simulink model "sm_car"  (R2025a)
settings: Solver=ode23t  StartTime=0.0  StopTime=400  MaxStep=0.4  RelTol=1e-3  AbsTol=1e-3  EnableMultiTasking=on
PreLoadFcn:
  | % Due to usability issue in Repeating Sequence block
  | warning('off','Simulink:Masking:Invalid');
  | 
  | % Eliminate unnecessary warnings in inactive variants
  | % Warnings generated only if you click through inactive variant
  | warning('off','MATLAB:nonExistentField');
  | warning('off','Simulink:Parameters:BlkParamUndefined');
PostLoadFcn:
  | set_param([bdroot '/Vehicle'],'popup_trailer','Off')
  | warning('off','sm:sli:setup:compile:LocalSolverNotSupported')
  | %sm_car_config_maneuver(bdroot,'WOT Braking');
  | sm_car_config_vehicle(bdroot,'false');
  | sm_car_config_logging(bdroot);
InitFcn:
  | sm_car_config_camera;
  | Vehicle = sm_car_vehcfg_checkConfig(Vehicle);
  | sm_car_check_tire_model(bdroot);
StartFcn:
  | tic;
StopFcn:
  | Elapsed_Sim_Time = toc;
  | % disp(['Elapsed Sim Time = ' num2str(Elapsed_Sim_Time)]);
undefined symbols (not defined in the file): Axle1D, AxleIn, Camera, Control, Driver, Free, Init, Maneuver, Pedal, RaceFix, RaceSpin, Scene, ShaftL1, ShaftL2, ShaftR1, ShaftR2, Soft, Stiff, Visual, X, xy_data_car_side, Y, Z
libraries: sm_lib x1546, nesl_utility x528, fl_lib x480, SimscapeFluids_lib x61, sdl_lib x49, simulink x29, ee_lib x7, simulink_extras x6, Linkage_Systems x4, Tire_1x2x x4, AntiRollBar_Systems x2, Linkage_Decoupled x2
(part 5 of 79)

== system sm_car/Controller/TrqVec 4Motor/Power_TqVec ==
  In Bus Element6 : Inport  PortName=DrvBus  Element=rAccelPedal
  In Bus Element2 : Inport  PortName=DrvBus  Element=aSteerWheel
  In Bus Element3 : Inport  PortName=DrvBus  Element=rBrakePedal
  In Bus Element : Inport  Port=2  PortName=VehBus  Element=Chassis.Body.CG.vx
  In Bus Element1 : Inport  Port=2  PortName=VehBus  Element=Power.MotorL2.w
  In Bus Element8 : Inport  Port=2  PortName=VehBus  Element=Power.MotorR2.w
  In Bus Element5 : Inport  Port=2  PortName=VehBus  Element=World.nYaw
  Bus Creator : BusCreator  Inputs=5
  Constant : Constant  Value=Control.trq_ratio_front
  Constant2 : Constant  Value=1-Control.trq_ratio_front
  Gain1 : Gain  Gain=1600
  Gain3 : Gain  Gain=0.5
  Gain4 : Gain  Gain=0.5
  Product : Product
  Product1 : Product
  Rate Limiter : RateLimiter  RisingSlewLimit=300  FallingSlewLimit=-5000  SampleTimeMode=inherited
  Torque Vectoring : Subsystem  mask(Torque Vectoring, Rear Wheels){vx_enable=Control.vx_enable, aSteerWheel_enable=Control.aSteerWheel_enable, aStr_to_aWhl=Control.aStr_to_aWhl, max_torque_delta=Control.max_torque_delta, P=Control.pGain, I=Control.iGain}
      mask prompts: vx_enable "Speed to enable (m/s)"; aSteerWheel_enable "Steering wheel angle to enable (rad)"; aStr_to_aWhl "Steering Ratio (Wheel/Steering Wheel)"; max_torque_delta "Max Torque Split (N*m)"; P "Simulink:masks:ProportionalP_MP"; I "Simulink:masks:IntegralI_MP"
      mask help: Basic torque vectoring algorithm which applies opposing offsets to the commanded torque of the rear wheels based on the error between the vehicle slip angle and the angle of the steered wheels.
      mask TypeOptions vx_enable: Enable/Enable vx/const
      mask TypeOptions aSteerWheel_enable: Enable/const/Value
      mask TypeOptions aStr_to_aWhl:
      | Vehicle Slip Angle Error/Steering Wheel
      | to Driving Wheel/Gain
      mask TypeOptions max_torque_delta: Max Delta Torque/Value
      mask TypeOptions P: PID Controller/P
      mask TypeOptions I: PID Controller/I
      mask DialogControl P Prompt: Proportional (P):
      mask DialogControl I Prompt: Integral (I):
  Power : Outport  VectorParamsAs1DForOutWhenUnconnected=off
  wires:
  Torque Vectoring/2(trqR2) -> Bus Creator/5  "MMotorR2Demand"
  Torque Vectoring/1(trqL2) -> Bus Creator/4  "MMotorL2Demand"
  In Bus Element3/1 -> Torque Vectoring/7(rBrake)
  In Bus Element5/1 -> Torque Vectoring/6(nYaw)
  In Bus Element8/1 -> Torque Vectoring/5(wR2)
  In Bus Element1/1 -> Torque Vectoring/4(wL2)
  In Bus Element2/1 -> Torque Vectoring/3(aSteerWheel)
  In Bus Element/1 -> Torque Vectoring/2(vx)
  Product1/1 -> Torque Vectoring/1(trqA2)
  Bus Creator/1 -> Power/1  "Power"
  Gain4/1 -> Bus Creator/3  "MMotorR1Demand"
  Gain3/1 -> Bus Creator/2  "MMotorL1Demand"
  Product/1 -> Gain4/1, Gain3/1, Bus Creator/1  "MMotorA1Demand"
  Constant2/1 -> Product1/2
  Constant/1 -> Product/1
  Rate Limiter/1 -> Product/2, Product1/1
  In Bus Element6/1 -> Gain1/1
  Gain1/1 -> Rate Limiter/1

== system sm_car/Controller/TrqVec 4Motor/Spring Control ==
  VehBus : Inport
  In Bus Element : Inport  Port=2  PortName=Ctrl  Element=Axle1
  In Bus Element1 : Inport  Port=2  PortName=Ctrl  Element=Axle2
  Bus Creator : BusCreator  Inputs=4
  Bus Selector : BusSelector  OutputSignals=Chassis.Damper.L1,Chassis.Damper.R1,Chassis.Damper.L2,Chassis.Damper.R2
  Spring Control A1 : Subsystem  Variant=on  VariantControlMode=label  VariantControl=Choice  LabelModeActiveChoice=None  mask(Spring Control, One Axle){popup_spring_control=None, popup_gas_spring=Stiff}
      mask prompts: popup_spring_control "Spring Control"; popup_gas_spring "Gas Spring"
      mask help: Configurable spring control for left and right sides.
      mask init:
      | bh = gcb;
      | set_param(bh,'LabelModeActiveChoice',get_param(bh,'popup_spring_control'));
      | set_param([bh '/Hydropneumatic'],'popup_gas_spring',get_param(bh,'popup_gas_spring'));
      mask TypeOptions popup_spring_control: None | Hydropneumatic
      mask Callback popup_spring_control:
      | bh = gcb;
      | maskObj = Simulink.Mask.get(bh); % Get the mask object of the current block
      | psg_h   = maskObj.getParameter('popup_gas_spring'); % Get the parameter to hide
      | 
      | % Check the value of ControlParam
      | controlParamValue = get_param(bh, 'popup_spring_control');
      | 
      | psg_h.Visible  = 'off';
      | 
      | if strcmp(controlParamValue, 'Hydropneumatic')
      |     psg_h.Visible  = 'on';
      | else
      |     psg_h.Visible  = 'off';
      | end
      mask TypeOptions popup_gas_spring: Stiff | Soft
      mask Display: disp(' ')
  Spring Control A2 : Subsystem  Variant=on  VariantControlMode=label  VariantControl=Choice  LabelModeActiveChoice=None  mask(Spring Control, One Axle){popup_spring_control=None, popup_gas_spring=Stiff}
      mask prompts: popup_spring_control "Spring Control"; popup_gas_spring "Gas Spring"
      mask help: Configurable spring control for left and right sides.
      mask init:
      | bh = gcb;
      | set_param(bh,'LabelModeActiveChoice',get_param(bh,'popup_spring_control'));
      | set_param([bh '/Hydropneumatic'],'popup_gas_spring',get_param(bh,'popup_gas_spring'));
      mask TypeOptions popup_spring_control: None | Hydropneumatic
      mask Callback popup_spring_control:
      | bh = gcb;
      | maskObj = Simulink.Mask.get(bh); % Get the mask object of the current block
      | psg_h   = maskObj.getParameter('popup_gas_spring'); % Get the parameter to hide
      | 
      | % Check the value of ControlParam
      | controlParamValue = get_param(bh, 'popup_spring_control');
      | 
      | psg_h.Visible  = 'off';
      | 
      | if strcmp(controlParamValue, 'Hydropneumatic')
      |     psg_h.Visible  = 'on';
      | else
      |     psg_h.Visible  = 'off';
      | end
      mask TypeOptions popup_gas_spring: Stiff | Soft
      mask Display: disp(' ')
  Spring : Outport
  wires:
  VehBus/1 -> Bus Selector/1
  Spring Control A1/1(L) -> Bus Creator/1  "L1"
  Bus Selector/1 -> Spring Control A1/1(mL)  "<L1>"
  Bus Selector/2 -> Spring Control A1/2(mR)  "<R1>"
  Bus Selector/3 -> Spring Control A2/1(mL)  "<L2>"
  Bus Selector/4 -> Spring Control A2/2(mR)  "<R2>"
  Bus Creator/1 -> Spring/1  "Spring"
  Spring Control A1/2(R) -> Bus Creator/2  "R1"
  Spring Control A2/1(L) -> Bus Creator/3  "L2"
  Spring Control A2/2(R) -> Bus Creator/4  "R2"
  In Bus Element/1 -> Spring Control A1/3(Inp)
  In Bus Element1/1 -> Spring Control A2/3(Inp)

== system sm_car/Controller/TrqVec 4Motor/Susp ==
  aSteerWheel : Inport
  vx : Inport  Port=2
  Bus Creator1 : BusCreator  Inputs=1
  Bus Creator3 : BusCreator  Inputs=1
  Steer Axle 1 : Subsystem
  Steer Axle 2 : Subsystem
  SuspA1 : Outport  VectorParamsAs1DForOutWhenUnconnected=off
  SuspA2 : Outport  Port=2  VectorParamsAs1DForOutWhenUnconnected=off
  wires:
  Steer Axle 2/1(Steer) -> Bus Creator3/1
  Bus Creator1/1 -> SuspA1/1  "SuspA1"
  Steer Axle 1/1(Steer) -> Bus Creator1/1
  aSteerWheel/1 -> Steer Axle 1/1(aSteerWheel), Steer Axle 2/1(aSteerWheel)  "aSteerWheel"
  Bus Creator3/1 -> SuspA2/1  "SuspA2"
  vx/1 -> Steer Axle 2/2(vx), Steer Axle 1/2(vx)

== system sm_car/Driver/Closed Loop/Driver ==
  vx : Inport
  Ref : Inport  Port=2
  CurPose : Inport  Port=3
  Preview : Inport  Port=4
  Bus Creator5 : BusCreator  Inputs=4
  Bus Selector1 : BusSelector  OutputSignals=vTarget
  Bus Selector2 : BusSelector  OutputSignals=dist
  Constant9 : Constant  Value=0
  Cur Pose : Subsystem
  Filter Steer Cmd : TransferFcn  Denominator=[1/Driver.Lateral.fSteerCutoff.Value 1]
  Fwd Rev : Subsystem
  Lateral Driver : Subsystem  Variant=on  VariantControlMode=label  VariantControl=Choice  LabelModeActiveChoice=Stanley  mask{Lateral=Driver.Lateral, VariantLabel=Driver.Lateral.class.Value}
      mask prompts: Lateral "Lateral Driver Parameters (structure)"; VariantLabel "Variant Label"
      mask init:
      | curblk = gcb;
      | 
      | % Set variant for this block 
      | set_param(curblk,'LabelModeActiveChoice',VariantLabel);
  Longitudinal Driver : Subsystem  mask(Longitudinal Driver (Velocity-tracking Controller)){SPEED_LOOKAHEAD_TIME=Driver.Long.FFLookahead.Value, C_ROLLING_RESISTANCE_COEFF=Driver.Long.NRollingResistance.Value, ROAD_FRICTION_COEFF=Driver.Long.NRoadFriction.Value, mVehicle=Driver.Long.mVehicle.Value, gGravity=Driver.Long.gGravity.Value, FTractive=Driver.Long.FTractive.Value, KP_SPEED=Driver.Long.Kp.Value, KI_SPEED=Driver.Long.Ki.Value, MAX_ACCEL_MPS2=Driver.Long.gMaxAccel.Value, MAX_DECEL_MPS2=Driver.Long.gMaxDecel.Value, Cdrag=Vehicle.Chassis.Aero.CD.Value, rho_air=Vehicle.Chassis.Aero.rho_air.Value, ARef=Vehicle.Chassis.Aero.ARef.Value}
      mask prompts: SPEED_LOOKAHEAD_TIME "Lookahead time (s)"; C_ROLLING_RESISTANCE_COEFF "Rolling resistance coefficient"; ROAD_FRICTION_COEFF "Road friction coefficient"; mVehicle "Total Vehicle mass (kg)"; gGravity "Gravity (m/s)"; FTractive "Tractive Force (N)"; KP_SPEED "Proportional gain, Kp"; KI_SPEED "Integral gain, Ki"; MAX_ACCEL_MPS2 "Max acceleration (m/s^2, positive number))"; MAX_DECEL_MPS2 "Max deceleration (m/s^2, must be negative)"; Cdrag "Drag coefficient"; rho_air "Density of air (kg/m^3)"; ARef "Frontal Area (m^2)"
      mask help: Implements a PI controller with feedforward for velocity tracking.
      mask DialogControl cont_feedforward Prompt: Feed-Forward Controller parameters
      mask DialogControl cont_feedback Prompt: Feedback Controller parameters
      mask DialogControl cont_drag Prompt: Drag
  Ref Pose and Distance : Subsystem
  Transfer Fcn : TransferFcn  Denominator=[1/(Driver.Long.fAccelCutoff.Value) 1]
  Transfer Fcn1 : TransferFcn  Denominator=[1/(Driver.Long.fBrakeCutoff.Value) 1]
  DrvBus : Outport  VectorParamsAs1DForOutWhenUnconnected=off
  wires:
  Bus Selector2/1 -> Longitudinal Driver/4(Distance)  "<dist>"
  Fwd Rev/2(vxFwRv) -> Longitudinal Driver/3(vx)
  Bus Selector1/1 -> Fwd Rev/2(vT)  "<vTarget>"
  Ref Pose and Distance/2(Dist) -> Lateral Driver/2(Distance)
  Preview/1 -> Longitudinal Driver/1(Preview), Lateral Driver/5(Preview)
  Lateral Driver/1(steeringAngle) -> Filter Steer Cmd/1
  Fwd Rev/1(dir) -> Longitudinal Driver/2(dir), Lateral Driver/6(Direction)
  vx/1 -> Fwd Rev/1(vx), Lateral Driver/4(v_x)
  Cur Pose/1(CurPose) -> Lateral Driver/3(currentPose)
  CurPose/1 -> Cur Pose/1(Cur)
  Constant9/1 -> Longitudinal Driver/5(current_slope_rad)
  Bus Creator5/1 -> DrvBus/1  "DrvBus"
  Longitudinal Driver/1(AccelCmd) -> Transfer Fcn/1
  Longitudinal Driver/2(DecelCmd) -> Transfer Fcn1/1
  Transfer Fcn1/1 -> Bus Creator5/4  "rBrakePedal"
  Transfer Fcn/1 -> Bus Creator5/3  "rAccelPedal"
  Ref/1 -> Bus Creator5/1, Bus Selector2/1, Bus Selector1/1, Ref Pose and Distance/1(Ref)
  Ref Pose and Distance/1(RefPose) -> Lateral Driver/1(referencePose)
  Filter Steer Cmd/1 -> Bus Creator5/2  "aSteerWheel"

== system sm_car/Driver/Closed Loop/Driver Override ==
  In : Inport
  None : Subsystem  VariantControl=None
  Override : Subsystem  VariantControl=Override
  DrvBus : Outport

== system sm_car/Driver/Closed Loop/Maneuver ==
  note: Fwd or
      | Rev
  VehBus : Inport
  Override : Inport  Port=2
  Abs : Abs  ZeroCross=off  SaturateOnIntegerOverflow=off
  Bus Creator : BusCreator  Inputs=7
  Bus Creator1 : BusCreator  Inputs=5
  Bus Selector : BusSelector  OutputSignals=World.x,World.y,World.z,World.aRoll,World.aPitch,World.aYaw,Chassis.Body.CG.vx
  Bus Selector1 : BusSelector  OutputSignals=x,y,z,vx
  Bus Selector2 : BusSelector  OutputSignals=Chassis.Body.CG.vx
  Bus Selector3 : BusSelector  OutputSignals=y,x,nLap,ayaw
  Constant : Constant  Value=-1
  Constant6 : Constant  Value=Maneuver.Trajectory.xTrajectory.Value
  Constant8 : Constant  Value=Maneuver.Trajectory.aYaw.Value
  Count Lap : Subsystem
  MATLAB Function : MATLAB Function  SystemSampleTime=0.1  mask{nPreviewPoints=Maneuver.nPreviewPoints.Value}
      mask prompts: nPreviewPoints "Number of Preview Points"
  Max Lateral Distance (m) : Constant  Value=Maneuver.xMaxLat.Value
  Memory : Memory  InitialCondition=-1
  Min Target Speed (m/s) : Constant  Value=Maneuver.vMinTarget.Value
  Mux : Mux  Inputs=3
  Mux1 : Mux  Inputs=3
  PoseTarget Visual : Subsystem
  Switch : Switch  Criteria=u2 > Threshold  SaturateOnIntegerOverflow=off  InputSameDT=off
  Target Speed Gain : Constant  Value=Maneuver.vGain.Value
  Window of Points to Check : Constant  Value=10
  preview distance : Lookup_n-D  NumberOfTableDimensions=1  BreakpointsForDimension1=Maneuver.xPreview.v.Value  Table=Maneuver.xPreview.x.Value  InternalRulePriority=Speed  RndMeth=Simplest
  vx override : Subsystem
  window only : Constant  Value=0
  x override : Subsystem
  y override : Subsystem
  z override : Subsystem
  vx : Outport  VectorParamsAs1DForOutWhenUnconnected=off
  Ref : Outport  Port=2  VectorParamsAs1DForOutWhenUnconnected=off
  CurPose : Outport  Port=3  VectorParamsAs1DForOutWhenUnconnected=off
  Preview : Outport  Port=4  VectorParamsAs1DForOutWhenUnconnected=off
  simres : Outport  Port=5  VectorParamsAs1DForOutWhenUnconnected=off
  wires:
  MATLAB Function/14(pp_preview_speed_pts) -> Bus Creator1/5  "pp_preview_speed_pts"
  MATLAB Function/1(ref_z) -> PoseTarget Visual/1(ref_z)
  Bus Selector3/4 -> PoseTarget Visual/5(ref_ayaw)  "<ayaw>"
  Bus Selector3/3 -> PoseTarget Visual/4(Lap Count)  "<nLap>"
  Bus Selector3/2 -> PoseTarget Visual/3(ref_x)  "<x>"
  Bus Selector3/1 -> PoseTarget Visual/2(ref_y)  "<y>"
  Count Lap/1(lapC) -> Bus Creator/1  "nLap"
  Bus Selector2/1 -> vx/1  "<vx>"
  VehBus/1 -> Bus Selector/1, Bus Selector2/1
  Bus Creator1/1 -> Preview/1  "lookahead"
  MATLAB Function/13(pp_preview_dist_pts) -> Bus Creator1/4  "pp_preview_dist_pts"
  MATLAB Function/12(pp_preview_yaw_pts) -> Bus Creator1/3  "pp_preview_yaw_pts"
  MATLAB Function/11(pp_preview_y_pts) -> Bus Creator1/2  "pp_preview_y_pts"
  MATLAB Function/10(pp_preview_x_pts) -> Bus Creator1/1  "pp_preview_x_pts"
  MATLAB Function/7(ld) -> Bus Creator/7  "latdev"
  Min Target Speed (m/s)/1 -> MATLAB Function/12(minSpd)
  Target Speed Gain/1 -> MATLAB Function/13(speedGain)
  Max Lateral Distance (m)/1 -> MATLAB Function/11(maxld)
  Bus Selector/1 -> Mux/1  "<x>"
  Bus Selector/6 -> Mux1/3  "<aYaw>"
  Bus Selector/4 -> Mux1/1  "<aRoll>"
  Constant8/1 -> MATLAB Function/8(yaw)
  Bus Selector/7 -> Abs/1  "<vx>"
  Mux1/1 -> MATLAB Function/2(q)
  Bus Selector/5 -> Mux1/2  "<aPitch>"
  Constant6/1 -> MATLAB Function/9(dist)
  Mux/1 -> MATLAB Function/1(p)
  Bus Selector/3 -> Mux/3  "<z>"
  y override/1(y_ovr) -> MATLAB Function/4(posy)
  Bus Selector/2 -> Mux/2  "<y>"
  MATLAB Function/3(ref_x) -> Bus Creator/3  "x"
  x override/1(x_ovr) -> MATLAB Function/3(posx)
  MATLAB Function/8(cp) -> CurPose/1  "CurPose"
  preview distance/1 -> MATLAB Function/10(pd)
  MATLAB Function/4(ref_y) -> Bus Creator/4  "y"
  MATLAB Function/5(ref_ayaw) -> Bus Creator/5  "ayaw"
  MATLAB Function/2(ad) -> Count Lap/1(ad), Bus Creator/2  "dist"
  Bus Creator/1 -> Bus Selector3/1, Ref/1  "Reference"
  MATLAB Function/6(vTarget) -> Bus Creator/6  "vTarget"
  MATLAB Function/9(simres) -> simres/1
  Window of Points to Check/1 -> MATLAB Function/7(xywin)
  MATLAB Function/15(idx_ptMin) -> Memory/1
  Switch/1 -> MATLAB Function/14(idx_ptMin_prev)
  Constant/1 -> Switch/3
  window only/1 -> Switch/2
  Memory/1 -> Switch/1
  z override/1(z_ovr) -> MATLAB Function/5(posz)
  Override/1 -> Bus Selector1/1
  Bus Selector1/4 -> vx override/1(vx)  "<vx>"
  vx override/1(vx_ovr) -> MATLAB Function/6(speed)
  Bus Selector1/3 -> z override/1(z)  "<z>"
  Bus Selector1/2 -> y override/1(y)  "<y>"
  Bus Selector1/1 -> x override/1(x)  "<x>"
  Abs/1 -> preview distance/1

== system sm_car/Driver/Closed Loop/Override ==
  "dist " : Inport
  "Obs " : Inport  Port=2
  None : Subsystem  VariantControl=None  mask(No Driver Override){override=Scene.Mallory_Park_Obstacle.Override}
      mask prompts: override "Override parameters (structure)"
      mask help: Driver commands are not overridden, regardless of inputs to subsystem.
  " Ovr" : Outport  VectorParamsAs1DForOutWhenUnconnected=off

== system sm_car/Driver/Closed Loop/Scopes ==
  <vx> : Inport
  Ref : Inport  Port=2
  CurPose : Inport  Port=3
  DrvBus : Inport  Port=4
  Bus Selector : BusSelector  OutputSignals=vTarget
  Bus Selector1 : BusSelector  OutputSignals=aSteerWheel,rAccelPedal,rBrakePedal
  Compare vx to Target : Scope  NumInputPorts=2
      settings: ActiveDisplayYMinimum=-4.79181  ActiveDisplayYMaximum=0.54534
  RefPose : Scope
      settings: ActiveDisplayYMinimum=-598.75829  ActiveDisplayYMaximum=469.37365
  Scope1 : Scope  NumInputPorts=3
      settings: ActiveDisplayYMinimum=-1.19495  ActiveDisplayYMaximum=0.13277  DataLoggingVariableName=ScopeData2
  wires:
  DrvBus/1 -> Bus Selector1/1
  Bus Selector1/1 -> Scope1/1  "<aSteerWheel>"
  Bus Selector1/2 -> Scope1/2  "<rAccelPedal>"
  <vx>/1 -> Compare vx to Target/1
  Bus Selector1/3 -> Scope1/3  "<rBrakePedal>"
  CurPose/1 -> RefPose/1
  Bus Selector/1 -> Compare vx to Target/2  "<vTarget>"
  Ref/1 -> Bus Selector/1

== system sm_car/Driver/Open Loop/Open Loop ==
  Bus Creator : BusCreator  Inputs=7
  Bus Creator5 : BusCreator  Inputs=4
  Constant : Constant  Value=10000
  Constant{1..6} (6 alike) : Constant  Value=0
  Input Sequence Accel Pedal : simulink/Sources/Repeating Sequence  rep_seq_t=Maneuver.Accel.t.Value  rep_seq_y=Maneuver.Accel.rPedal.Value
  Input Sequence Brake Pedal : simulink/Sources/Repeating Sequence  rep_seq_t=Maneuver.Brake.t.Value  rep_seq_y=Maneuver.Brake.rPedal.Value
  "Input Sequence Steering Wheel " : simulink/Sources/Repeating Sequence  rep_seq_t=Maneuver.Steer.t.Value  rep_seq_y=Maneuver.Steer.aWheel.Value
  DrvBus : Outport  VectorParamsAs1DForOutWhenUnconnected=off
  wires:
  Constant6/1 -> Bus Creator/7  "nLap"
  Constant/1 -> Bus Creator/1  "dist"
  Bus Creator/1 -> Bus Creator5/1  "Reference"
  Constant4/1 -> Bus Creator/5  "vTarget"
  Constant3/1 -> Bus Creator/4  "ayaw"
  Constant2/1 -> Bus Creator/3  "y"
  Constant5/1 -> Bus Creator/6  "latdev"
  Constant1/1 -> Bus Creator/2  "x"
  Input Sequence Accel Pedal/1 -> Bus Creator5/3  "rAccelPedal"
  "Input Sequence Steering Wheel "/1 -> Bus Creator5/2  "aSteerWheel"
  Input Sequence Brake Pedal/1 -> Bus Creator5/4  "rBrakePedal"
  Bus Creator5/1 -> DrvBus/1  "DrvBus"

== system sm_car/Road/Mu Scaling by Position/Scaling factors FL ==
  muX : Inport
  muY : Inport  Port=2
  s_LKX : Constant  Value=LKX
  s_LKY : Constant  Value=LKY
  s_LKYC : Constant  Value=LKYC
  s_LKZC : Constant  Value=LKZC
  s_LTR : Constant  Value=LTR
  scaling_vector : Mux  Inputs=7
  scaling : Outport  VectorParamsAs1DForOutWhenUnconnected=off
  wires:
  muX/1 -> scaling_vector/1
  s_LKX/1 -> scaling_vector/2
  muY/1 -> scaling_vector/3
  s_LKY/1 -> scaling_vector/4
  s_LKYC/1 -> scaling_vector/5
  s_LTR/1 -> scaling_vector/6
  s_LKZC/1 -> scaling_vector/7
  scaling_vector/1 -> scaling/1

== system sm_car/Road/Mu Scaling by Position/Scaling factors FR ==
  muX : Inport
  muY : Inport  Port=2
  s_LKX : Constant  Value=LKX
  s_LKY : Constant  Value=LKY
  s_LKYC : Constant  Value=LKYC
  s_LKZC : Constant  Value=LKZC
  s_LTR : Constant  Value=LTR
  scaling_vector : Mux  Inputs=7
  scaling : Outport  VectorParamsAs1DForOutWhenUnconnected=off
  wires:
  muX/1 -> scaling_vector/1
  s_LKX/1 -> scaling_vector/2
  muY/1 -> scaling_vector/3
  s_LKY/1 -> scaling_vector/4
  s_LKYC/1 -> scaling_vector/5
  s_LTR/1 -> scaling_vector/6
  s_LKZC/1 -> scaling_vector/7
  scaling_vector/1 -> scaling/1

== system sm_car/Road/Mu Scaling by Position/Scaling factors RL ==
  muX : Inport
  muY : Inport  Port=2
  s_LKX : Constant  Value=LKX
  s_LKY : Constant  Value=LKY
  s_LKYC : Constant  Value=LKYC
  s_LKZC : Constant  Value=LKZC
  s_LTR : Constant  Value=LTR
  scaling_vector : Mux  Inputs=7
  scaling : Outport  VectorParamsAs1DForOutWhenUnconnected=off
  wires:
  muX/1 -> scaling_vector/1
  s_LKX/1 -> scaling_vector/2
  muY/1 -> scaling_vector/3
  s_LKY/1 -> scaling_vector/4
  s_LKYC/1 -> scaling_vector/5
  s_LTR/1 -> scaling_vector/6
  s_LKZC/1 -> scaling_vector/7
  scaling_vector/1 -> scaling/1

== system sm_car/Road/Mu Scaling by Position/Scaling factors RR ==
  muX : Inport
  muY : Inport  Port=2
  s_LKX : Constant  Value=LKX
  s_LKY : Constant  Value=LKY
  s_LKYC : Constant  Value=LKYC
  s_LKZC : Constant  Value=LKZC
  s_LTR : Constant  Value=LTR
  scaling_vector : Mux  Inputs=7
  scaling : Outport  VectorParamsAs1DForOutWhenUnconnected=off
  wires:
  muX/1 -> scaling_vector/1
  s_LKX/1 -> scaling_vector/2
  muY/1 -> scaling_vector/3
  s_LKY/1 -> scaling_vector/4
  s_LKYC/1 -> scaling_vector/5
  s_LTR/1 -> scaling_vector/6
  s_LKZC/1 -> scaling_vector/7
  scaling_vector/1 -> scaling/1

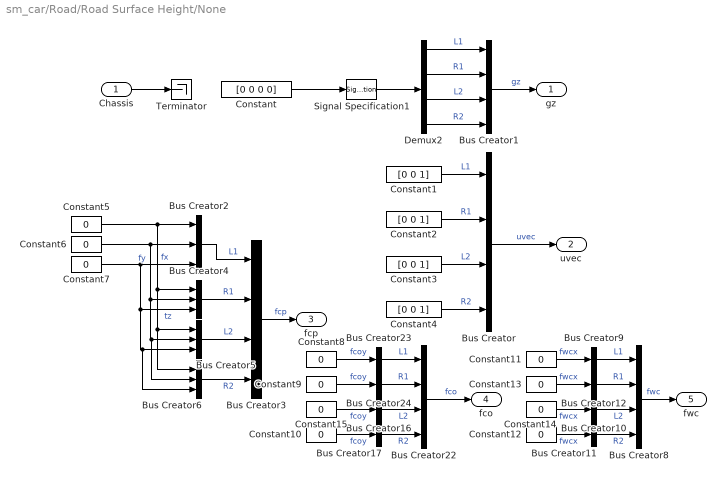
== system sm_car/Road/Road Surface Height/None ==
  Chassis : Inport
  Bus Creator{,1,3,8,22} (5 alike) : BusCreator  Inputs=4
  Bus Creator{9..12,16..17,23..24} (8 alike) : BusCreator  Inputs=1
  Bus Creator{2,4..6} (4 alike) : BusCreator  Inputs=3
  Constant : Constant  Value=[0 0 0 0]
  Constant{1..4} (4 alike) : Constant  Value=[0 0 1]
  Constant{5..15} (11 alike) : Constant  Value=0
  Demux2 : Demux
  Signal Specification1 : SignalSpecification  Unit=m
  Terminator : Terminator
  gz : Outport  VectorParamsAs1DForOutWhenUnconnected=off
  uvec : Outport  Port=2  VectorParamsAs1DForOutWhenUnconnected=off
  fcp : Outport  Port=3  VectorParamsAs1DForOutWhenUnconnected=off
  fco : Outport  Port=4  VectorParamsAs1DForOutWhenUnconnected=off
  fwc : Outport  Port=5  VectorParamsAs1DForOutWhenUnconnected=off
  wires:
  Bus Creator24/1 -> Bus Creator22/2  "R1"
  Constant13/1 -> Bus Creator12/1  "fwcx"
  Constant14/1 -> Bus Creator10/1  "fwcx"
  Constant12/1 -> Bus Creator11/1  "fwcx"
  Bus Creator12/1 -> Bus Creator8/2  "R1"
  Bus Creator10/1 -> Bus Creator8/3  "L2"
  Constant11/1 -> Bus Creator9/1  "fwcx"
  Bus Creator23/1 -> Bus Creator22/1  "L1"
  Bus Creator17/1 -> Bus Creator22/4  "R2"
  Constant10/1 -> Bus Creator17/1  "fcoy"
  Bus Creator9/1 -> Bus Creator8/1  "L1"
  Constant9/1 -> Bus Creator24/1  "fcoy"
  Bus Creator8/1 -> fwc/1  "fwc"
  Bus Creator22/1 -> fco/1  "fco"
  Constant15/1 -> Bus Creator16/1  "fcoy"
  Bus Creator16/1 -> Bus Creator22/3  "L2"
  Bus Creator11/1 -> Bus Creator8/4  "R2"
  Constant8/1 -> Bus Creator23/1  "fcoy"
  Bus Creator/1 -> uvec/1  "uvec"
  Constant4/1 -> Bus Creator/4  "R2"
  Constant1/1 -> Bus Creator/1  "L1"
  Constant2/1 -> Bus Creator/2  "R1"
  Constant3/1 -> Bus Creator/3  "L2"
  Demux2/3 -> Bus Creator1/3  "L2"
  Demux2/4 -> Bus Creator1/4  "R2"
  Demux2/2 -> Bus Creator1/2  "R1"
  Bus Creator1/1 -> gz/1  "gz"
  Signal Specification1/1 -> Demux2/1
  Demux2/1 -> Bus Creator1/1  "L1"
  Constant/1 -> Signal Specification1/1
  Chassis/1 -> Terminator/1
  Constant5/1 -> Bus Creator6/1, Bus Creator5/1, Bus Creator4/1, Bus Creator2/1  "fx"
  Constant6/1 -> Bus Creator6/2, Bus Creator5/2, Bus Creator4/2, Bus Creator2/2  "fy"
  Constant7/1 -> Bus Creator6/3, Bus Creator5/3, Bus Creator4/3, Bus Creator2/3  "tz"
  Bus Creator2/1 -> Bus Creator3/1  "L1"
  Bus Creator3/1 -> fcp/1  "fcp"
  Bus Creator4/1 -> Bus Creator3/2  "R1"
  Bus Creator5/1 -> Bus Creator3/3  "L2"
  Bus Creator6/1 -> Bus Creator3/4  "R2"

== system sm_car/Vehicle/Trailer/None ==
  note: Ports deliberately not connected. They are necessary for unit tests, but not necessary here.
  "RdBus " : Inport
  "DrvBus " : Inport  Port=2
  "CtrlBus " : Inport  Port=3
  Ground : Ground
  Reference Frame : sm_lib/Frames and Transforms/Reference Frame
  Terminator : Terminator
  Terminator1 : Terminator
  Terminator2 : Terminator
  " C" : PMIOPort  Side=Left
  " W" : PMIOPort  Port=2  Side=Left
  " Hitch" : PMIOPort  Port=3  Side=Right
  " VehBus" : Outport  VectorParamsAs1DForOutWhenUnconnected=off
  wires:
  "RdBus "/1 -> Terminator/1
  "DrvBus "/1 -> Terminator1/1
  "CtrlBus "/1 -> Terminator2/1
  Ground/1 -> " VehBus"/1
  connections:
  " Hitch"/RConn1 -- Reference Frame/RConn1

== system sm_car/Vehicle/Vehicle/Body to World ==
  Free : Subsystem  VariantControl=Free  mask(Body to World){Init=Init.Chassis, SpecifyPosTarget=on}
      mask prompts: Init "Initial Values"; SpecifyPosTarget "Specify Position Target"
      mask help: Models the connection between the vehicle body and world. Permits 6 degrees of freedom and sets the initial position, orientation, and speed of the vehicle body.
      mask init:
      | initial_aveh = [Init.aChassis.Value(3) Init.aChassis.Value(2) Init.aChassis.Value(1)];
      | rotmat_ypr = sm_car_yawpitchroll_to_rotmat(Init.aChassis.Value(3),Init.aChassis.Value(2),Init.aChassis.Value(1));
      | initial_vveh = rotmat_ypr*(Init.vChassis.Value)';
      | 
      | sptState = get_param(gcb,'SpecifyPosTarget');
      | 
      | set_param([gcb '/Body World Joint'],...
      |         'PxPositionTargetSpecify',sptState,...
      |         'PyPositionTargetSpecify',sptState,...
      |         'PzPositionTargetSpecify',sptState,...
      |         'SphPositionTargetSpecify',sptState,...
      |         'PxVelocityTargetSpecify',sptState,...
      |         'PyVelocityTargetSpecify',sptState,...
      |         'PzVelocityTargetSpecify',sptState,...
      |         'SphVelocityTargetSpecify',sptState...
      |         );
      mask Help: web('sm_car_doc_body_to_world.html')
  F : PMIOPort  Side=Left
  B : PMIOPort  Port=2  Side=Right
  World : Outport

== system sm_car/Vehicle/Vehicle/Brakes ==
  "DrvBus " : Inport
  "CtrlBus " : Inport  Port=2
  PedalAbstract DiscDisc : Subsystem  Tag=PublishSubsystem  VariantControl=PedalAbstract_DiscDisc  mask(Disc Brakes, Pedal Input){brk_pad_rad_a1=Brakes.Axle1.DiscAndPad.lMeanRadius.Value, brk_pad_rad_a2=Brakes.Axle2.DiscAndPad.lMeanRadius.Value, brk_cyl_bore_a1=Brakes.Axle1.Caliper.lCylinderDiameter.Value, brk_cyl_bore_a2=Brakes.Axle2.Caliper.lCylinderDiameter.Value, brk_n_pads_a1=Brakes.Axle1.DiscAndPad.NPads.Value, brk_n_pads_a2=Brakes.Axle2.DiscAndPad.NPads.Value, brk_mu_static_a1=Brakes.Axle1.DiscAndPad.rMuStatic.Value, brk_mu_static_a2=Brakes.Axle2.DiscAndPad.rMuStatic.Value, brk_mu_kin_a1=Brakes.Axle1.DiscAndPad.rMuKinetic.Value, brk_mu_kin_a2=Brakes.Axle2.DiscAndPad.rMuKinetic.Value, brk_trans_vel_a1=Brakes.Axle1.DiscAndPad.nTransition.Value, brk_trans_vel_a2=Brakes.Axle2.DiscAndPad.nTransition.Value, brk_visc_coef_a1=Brakes.Axle1.DiscAndPad.dViscous.Value, brk_visc_coef_a2=Brakes.Axle2.DiscAndPad.dViscous.Value, brk_max_p_a1=Brakes.Axle1.Caliper.pMax.Value, brk_max_p_a2=Brakes.Axle2.Caliper.pMax.Value, brk_filt_a1=1/Brakes.Axle1.Caliper.fActuatorCutoff.Value, brk_filt_a2=1/Brakes.Axle2.Caliper.fActuatorCutoff.Value}
      mask help: Model braking system with disc brakes for two axles. Takes brake pedal travel as input, actuator dynamics modeled as a transfer function.
      mask TypeOptions brk_pad_rad_a1:
      | Disc
      | Brake
      | L1/r_mean | Disc
      | Brake
      | R1/r_mean
      mask TypeOptions brk_pad_rad_a2:
      | Disc
      | Brake
      | L2/r_mean | Disc
      | Brake
      | R2/r_mean
      mask TypeOptions brk_cyl_bore_a1:
      | Disc
      | Brake
      | L1/bore | Disc
      | Brake
      | R1/bore
      mask TypeOptions brk_cyl_bore_a2:
      | Disc
      | Brake
      | L2/bore | Disc
      | Brake
      | R2/bore
      mask TypeOptions brk_n_pads_a1:
      | Disc
      | Brake
      | L1/n_pads | Disc
      | Brake
      | R1/n_pads
      mask TypeOptions brk_n_pads_a2:
      | Disc
      | Brake
      | L2/n_pads | Disc
      | Brake
      | R2/n_pads
      mask TypeOptions brk_mu_static_a1:
      | Disc
      | Brake
      | L1/mu_static | Disc
      | Brake
      | R1/mu_static
      mask TypeOptions brk_mu_static_a2:
      | Disc
      | Brake
      | L2/mu_static | Disc
      | Brake
      | R2/mu_static
      mask TypeOptions brk_mu_kin_a1:
      | Disc
      | Brake
      | L1/mu_coulomb | Disc
      | Brake
      | R1/mu_coulomb
      mask TypeOptions brk_mu_kin_a2:
      | Disc
      | Brake
      | L2/mu_coulomb | Disc
      | Brake
      | R2/mu_coulomb
      mask TypeOptions brk_trans_vel_a1:
      | Disc
      | Brake
      | L1/brkwy_vel | Disc
      | Brake
      | R1/brkwy_vel
      mask TypeOptions brk_trans_vel_a2:
      | Disc
      | Brake
      | L2/brkwy_vel | Disc
      | Brake
      | R2/brkwy_vel
      mask TypeOptions brk_visc_coef_a1:
      | Disc
      | Brake
      | L1/visc_coef | Disc
      | Brake
      | R1/visc_coef
      mask TypeOptions brk_visc_coef_a2:
      | Disc
      | Brake
      | L2/visc_coef | Disc
      | Brake
      | R2/visc_coef
      mask TypeOptions brk_max_p_a1: Actuator L1/brk_max_p | Actuator R1/brk_max_p
      mask TypeOptions brk_max_p_a2: Actuator L2/brk_max_p | Actuator R2/brk_max_p
      mask TypeOptions brk_filt_a1: Actuator L1/brk_filt | Actuator R1/brk_filt
      mask TypeOptions brk_filt_a2: Actuator L2/brk_filt | Actuator R2/brk_filt
      mask DialogControl cont_brakes Prompt: Brakes
      mask DialogControl cont_brk_geom Prompt: Geometry
      mask DialogControl text_brakes_a1 Prompt: Axle 1
      mask DialogControl text_brakes_a2 Prompt: Axle 2
      mask DialogControl text_brakes_pad_rad Prompt: Mean Pad Radius (m)
      mask DialogControl text_brakes_cyl_bore Prompt: Cylinder Bore (m)
      mask DialogControl text_brakes_n_pads Prompt: Number of pads
      mask DialogControl cont_brk_frict Prompt: Friction
      mask DialogControl text_brakes_mu_static Prompt: Static Coeff. (0-1)
      mask DialogControl text_brakes_mu_kin Prompt: Kinetic Coeff. (0-1)
      mask DialogControl text_brakes_trans_vel Prompt: Trans. Velocity (rad/s)
      mask DialogControl text_brakes_visc_coef Prompt: Viscous (N*m/(rad/s))
      mask DialogControl cont_brk_act Prompt: Actuator
      mask DialogControl text_brakes_maxp Prompt: Max Pad Pressure (Pa)
      mask DialogControl text_brakes_filt Prompt: Time Constant (s)
      mask Display: image('sm_car_vehicle_brakes_pedal_IMAGE.png');
  L1 : PMIOPort  Side=Left
  R1 : PMIOPort  Port=2  Side=Right
  L2 : PMIOPort  Port=3  Side=Left
  R2 : PMIOPort  Port=4  Side=Right
  " OutB" : Outport  VectorParamsAs1DForOutWhenUnconnected=off

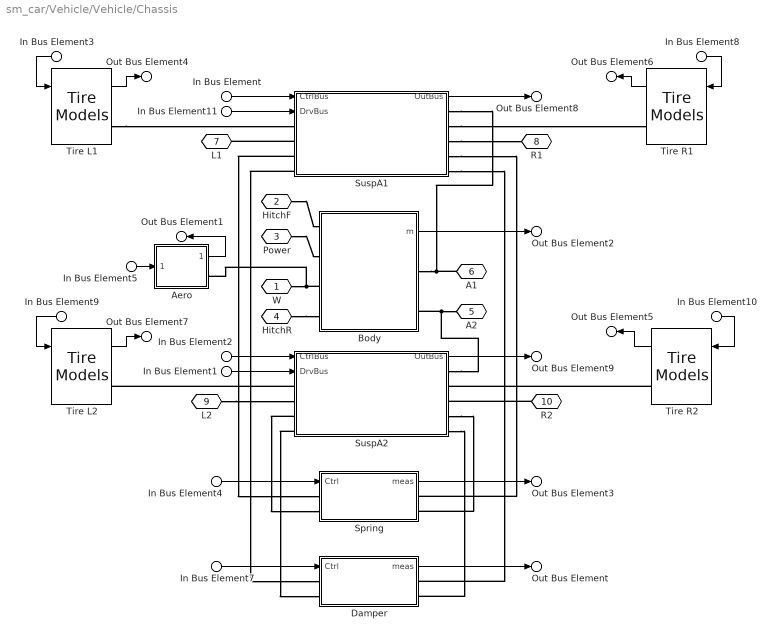
== system sm_car/Vehicle/Vehicle/Chassis ==
  In Bus Element11 : Inport  PortName=DrvBus
  In Bus Element1 : Inport  PortName=DrvBus
  In Bus Element3 : Inport  Port=2  PortName=RdBus  Element=L1
  In Bus Element8 : Inport  Port=2  PortName=RdBus  Element=R1
  In Bus Element10 : Inport  Port=2  PortName=RdBus  Element=R2
  In Bus Element9 : Inport  Port=2  PortName=RdBus  Element=L2
  In Bus Element5 : Inport  Port=2  PortName=RdBus  Element=fWindCar
  In Bus Element7 : Inport  Port=3  PortName=CtrlBus  Element=Damper
  In Bus Element : Inport  Port=3  PortName=CtrlBus  Element=SuspA1
  In Bus Element4 : Inport  Port=3  PortName=CtrlBus  Element=Spring
  In Bus Element2 : Inport  Port=3  PortName=CtrlBus  Element=SuspA2
  Aero : Subsystem  mask(Aerodynamic Load (Drag, Lift)){CL=Chassis.Aero.CL.Value, CD=Chassis.Aero.CD.Value, rho=Chassis.Aero.rho_air.Value, A=Chassis.Aero.ARef.Value, sCentreOfPressure=Chassis.Aero.sPressureCentre.Value, clr_hp=Visual.hp.clr, opc_hp=Visual.hp.opc, rad_hp=Visual.hp.rad}
      mask prompts: CL "Lift Coeff (-)"; CD "Drag Coeff (-)"; rho "Air Density (kg/m^3)"; A "Reference Area (m^2)"; sCentreOfPressure "Centre of Pressure [xyz] (m)"; clr_hp "Color [RGB]"; opc_hp "Opacity (0-1)"; rad_hp "Radius (m)"
      mask help: Models lift and drag on vehicle.
      mask TypeOptions clr_hp:
      | Vis
      | Center of Pressure/GraphicDiffuseColor
      mask TypeOptions opc_hp:
      | Vis
      | Center of Pressure/GraphicOpacity
      mask TypeOptions rad_hp:
      | Vis
      | Center of Pressure/SphereRadius
      mask DialogControl conv_vis Prompt: Visualization
  Body : Subsystem  mask(Body){hp_mount_a1=Chassis.Body.sAxle1.Value, hp_mount_a2=Chassis.Body.sAxle2.Value, hp_mount_power=Chassis.Body.sPower.Value, hp_chassis_cg=Chassis.Body.sCG.Value, hp_mount_hitchf=Chassis.Body.sHitchF.Value, hp_mount_hitchr=Chassis.Body.sHitchR.Value, chassis_mass=Chassis.Body.m.Value, chassis_inertia=Chassis.Body.J.Value, clr_chassis_hp_cg=Visual.hp.clr, opc_chassis_hp_cg=Visual.hp.opc, size_chassis_hp_cg=Visual.hp.rad, BodyGeometry=Chassis.Body.BodyGeometry, Passenger=Chassis.Body.Passenger, BodyLoad=Chassis.Body.BodyLoad}
      mask prompts: hp_mount_power "HP Power [xyz] (m)"; hp_chassis_cg "Chassis CG [xyz] (m)"; hp_mount_hitchf "Hitch Front [xyz] (m)"; hp_mount_hitchr "Hitch Rear [xyz] (m)"; chassis_mass "Mass (kg)"; chassis_inertia "Inertia [Ixx Iyy Izz]"; BodyGeometry "BodyGeometry (structure)"; Passenger "Passenger (structure)"; BodyLoad "BodyLoad (structure)"
      mask help: Vehicle body mass, inertia, and geometry.
      mask TypeOptions hp_mount_a1:
      | Transform
      | Mount A1/TranslationCartesianOffset
      mask TypeOptions hp_mount_a2:
      | Transform
      | Mount A2/TranslationCartesianOffset
      mask TypeOptions hp_mount_power:
      | Transform
      | Power Mount/TranslationCartesianOffset
      mask TypeOptions hp_chassis_cg:
      | Transform
      | Body CG/TranslationCartesianOffset
      mask TypeOptions hp_mount_hitchf:
      | Transform
      | Front Hitch/TranslationCartesianOffset
      mask TypeOptions hp_mount_hitchr:
      | Transform
      | Rear Hitch/TranslationCartesianOffset
      mask TypeOptions chassis_mass:
      | Body Mass
      | and Inertia/Mass
      mask TypeOptions chassis_inertia:
      | Body Mass
      | and Inertia/MomentsOfInertia
      mask TypeOptions clr_chassis_hp_cg:
      | Body Mass
      | and Inertia/GraphicDiffuseColor | Vis HP Mount A1/GraphicDiffuseColor | Vis HP Hitch/GraphicDiffuseColor
      mask TypeOptions opc_chassis_hp_cg:
      | Body Mass
      | and Inertia/GraphicOpacity | Vis HP Mount A1/GraphicOpacity | Vis HP Hitch/GraphicOpacity
      mask TypeOptions size_chassis_hp_cg:
      | Body Mass
      | and Inertia/SphereRadius | Vis HP Mount A1/SphereRadius | Vis HP Hitch/SphereRadius
      mask DialogControl cont_chassis Prompt: Chassis
      mask DialogControl text_chassis_mount_hp_blank Prompt: [xyz] (m)
      mask DialogControl text_chassis_a1 Prompt: Axle 1
      mask DialogControl text_chassis_a2 Prompt: Axle 2
      mask DialogControl text_chassis_hp_mount Prompt: HP Mount
      mask DialogControl cont_chassis_vis Prompt: Visualization
      mask DialogControl text_chassis_vis_clr Prompt: Color [RGB]
      mask DialogControl text_chassis_vis_opc Prompt: Opacity (0-1)
      mask DialogControl text_chassis_vis_size Prompt: Size [xyz] (m)
      mask DialogControl text_chassis_vis_hp Prompt: Hardpoints
      mask DialogControl cont_body_geometry Prompt: Body
      mask Display:
      | % Get image from BodyGeometry.class
      | % (active choice for Body Geometry subsystem)
      | temp_veh_bg_class = lower(get_param([gcb '/Body Geometry'],'LabelModeActiveChoice'));
      | 
      | imagestr = (['sm_car_body_' temp_veh_bg_class '.png']);
      | if(~exist(imagestr))
      |     imagestr = ['sm_car_body_default.png'];
      | end
      | 
      | image(imagestr);
  Damper : Subsystem  Tag=PublishSubsystem  Variant=on  VariantControlMode=label  VariantControl=Variant1  LabelModeActiveChoice=Independent  mask(Variants for Dampers){Damper=Chassis.Damper, VariantLabel=Chassis.Damper.class.Value}
      mask prompts: Damper "Damper Parameters"; VariantLabel "Variant Label"
      mask help: Select option and provide parameters for left and right dampers on two axles. Option is chosen by string provided in Variant Label. The parameters for the selected option is contained in Dampers data structure.
      mask init:
      | curblk = gcb;
      | 
      | % Set variant for this block 
      | set_param(curblk,'LabelModeActiveChoice',VariantLabel);
      settings: AttributesFormatString=%<ActiveVariant>
      mask Display:
      | if(strcmp(get_param(gcb,'LabelModeActiveChoice'),'None'))
      |     disp(' ');
      | else
      |     image('sm_car_vehicle_chassis_damper_IMAGE.png');
      | end
  Spring : Subsystem  Tag=PublishSubsystem  Variant=on  VariantControlMode=label  VariantControl=Variant1  LabelModeActiveChoice=Independent  mask(Variants for Springs){Spring=Chassis.Spring, VariantLabel=Chassis.Spring.class.Value}
      mask prompts: Spring "Spring Parameters"; VariantLabel "Variant Label"
      mask help: Select option and provide parameters for left and right springs on two axles. Option is chosen by string provided in Variant Label. The parameters for the selected option is contained in Springs data structure.
      mask init:
      | curblk = gcb;
      | 
      | % Set variant for this block 
      | set_param(curblk,'LabelModeActiveChoice',VariantLabel);
      settings: AttributesFormatString=%<ActiveVariant>
      mask Display:
      | if(strcmp(get_param(gcb,'LabelModeActiveChoice'),'None'))
      |     disp(' ');
      | else
      |     image('sm_car_vehicle_chassis_spring_IMAGE.png');
      | end
  SuspA1 : Subsystem  Variant=on  VariantControlMode=label  VariantControl=Variant1  LabelModeActiveChoice=Linkage  mask(Suspension and Steering){Susp=Chassis.SuspA1, Init=Init.Axle1, VariantLabel=Chassis.SuspA1.class.Value}
      mask prompts: Susp "Suspension Parameters"; Init "Initial Values"; VariantLabel "Variant Label"
      mask help: Models suspension and optional steering system for one axle. Option is chosen by string provided in Variant Label. The parameters for the selected option are contained in Suspension Parameters data structure.
      mask init:
      | curblk = gcb;
      | 
      | % Set variant for this block 
      | set_param(curblk,'LabelModeActiveChoice',VariantLabel);
      settings: AttributesFormatString=%<LabelModeActiveChoice>
  SuspA2 : Subsystem  Variant=on  VariantControlMode=label  VariantControl=Variant1  LabelModeActiveChoice=Linkage  mask(Suspension and Steering){Susp=Chassis.SuspA2, Init=Init.Axle2, VariantLabel=Chassis.SuspA2.class.Value}
      mask prompts: Susp "Suspension Parameters"; Init "Initial Values"; VariantLabel "Variant Label"
      mask help: Models suspension and optional steering system for one axle. Option is chosen by string provided in Variant Label. The parameters for the selected option are contained in Suspension Parameters data structure.
      mask init:
      | curblk = gcb;
      | 
      | % Set variant for this block 
      | set_param(curblk,'LabelModeActiveChoice',VariantLabel);
      settings: AttributesFormatString=%<LabelModeActiveChoice>
  Tire L1 : Tire_1x2x/Tire Models  Tag=PublishSubsystem  VariantControl=Variant1  LabelModeActiveChoice=MFMbody  popup_leftRight=Left  tir_index=veh_index  Tire=Chassis.TireA1  VariantLabel=Chassis.TireA1.class.Value
      settings: AttributesFormatString=%<ActiveVariant>
  Tire L2 : Tire_1x2x/Tire Models  Tag=PublishSubsystem  VariantControl=Variant1  LabelModeActiveChoice=MFMbody  popup_leftRight=Left  tir_index=veh_index+10  Tire=Chassis.TireA2  VariantLabel=Chassis.TireA2.class.Value
      settings: AttributesFormatString=%<ActiveVariant>
  Tire R1 : Tire_1x2x/Tire Models  Tag=PublishSubsystem  VariantControl=Variant1  LabelModeActiveChoice=MFMbody  popup_leftRight=Right  tir_index=veh_index+4  Tire=Chassis.TireA1  VariantLabel=Chassis.TireA1.class.Value
      settings: AttributesFormatString=%<ActiveVariant>
  Tire R2 : Tire_1x2x/Tire Models  Tag=PublishSubsystem  VariantControl=Variant1  LabelModeActiveChoice=MFMbody  popup_leftRight=Right  tir_index=veh_index+14  Tire=Chassis.TireA2  VariantLabel=Chassis.TireA2.class.Value
      settings: AttributesFormatString=%<ActiveVariant>
  W : PMIOPort  Side=Right
  HitchF : PMIOPort  Port=2  Side=Right
  Power : PMIOPort  Port=3  Side=Right
  HitchR : PMIOPort  Port=4  Side=Left
  A2 : PMIOPort  Port=5  Side=Right
  A1 : PMIOPort  Port=6  Side=Left
  L1 : PMIOPort  Port=7  Side=Left
  R1 : PMIOPort  Port=8  Side=Right
  L2 : PMIOPort  Port=9  Side=Left
  R2 : PMIOPort  Port=10  Side=Right
  Out Bus Element4 : Outport  VectorParamsAs1DForOutWhenUnconnected=off  PortName=VehBus  Element=WhlL1
  Out Bus Element6 : Outport  VectorParamsAs1DForOutWhenUnconnected=off  PortName=VehBus  Element=WhlR1
  Out Bus Element5 : Outport  VectorParamsAs1DForOutWhenUnconnected=off  PortName=VehBus  Element=WhlR2
  Out Bus Element7 : Outport  VectorParamsAs1DForOutWhenUnconnected=off  PortName=VehBus  Element=WhlL2
  Out Bus Element1 : Outport  VectorParamsAs1DForOutWhenUnconnected=off  PortName=VehBus  Element=Aero
  Out Bus Element : Outport  VectorParamsAs1DForOutWhenUnconnected=off  PortName=VehBus  Element=Damper
  Out Bus Element3 : Outport  VectorParamsAs1DForOutWhenUnconnected=off  PortName=VehBus  Element=Spring
  Out Bus Element8 : Outport  VectorParamsAs1DForOutWhenUnconnected=off  PortName=VehBus  Element=SuspA1
  Out Bus Element9 : Outport  VectorParamsAs1DForOutWhenUnconnected=off  PortName=VehBus  Element=SuspA2
  Out Bus Element2 : Outport  VectorParamsAs1DForOutWhenUnconnected=off  PortName=VehBus  Element=Body
  wires:
  Body/1(m) -> Out Bus Element2/1
  In Bus Element5/1 -> Aero/1(fWind)
  Aero/1(meas) -> Out Bus Element1/1
  In Bus Element4/1 -> Spring/1("Ctrl ")
  In Bus Element7/1 -> Damper/1("Ctrl ")
  In Bus Element2/1 -> SuspA2/1("CtrlBus ")
  SuspA2/1(OutBus) -> Out Bus Element9/1
  In Bus Element1/1 -> SuspA2/2(DrvBus)
  In Bus Element/1 -> SuspA1/1("CtrlBus ")
  SuspA1/1(OutBus) -> Out Bus Element8/1
  In Bus Element11/1 -> SuspA1/2(DrvBus)
  Tire R2/1 -> Out Bus Element5/1
  In Bus Element9/1 -> Tire L2/1
  Tire L1/1 -> Out Bus Element4/1
  In Bus Element8/1 -> Tire R1/1
  Tire L2/1 -> Out Bus Element7/1
  In Bus Element10/1 -> Tire R2/1
  Tire R1/1 -> Out Bus Element6/1
  In Bus Element3/1 -> Tire L1/1
  Damper/1(" meas") -> Out Bus Element/1
  Spring/1(" meas") -> Out Bus Element3/1
  connections:
  HitchR/RConn1 -- Body/LConn4
  Power/RConn1 -- Body/LConn2
  SuspA2/RConn5 -- Damper/RConn2
  SuspA2/LConn4 -- Damper/LConn2
  SuspA2/RConn4 -- Spring/RConn2
  SuspA2/LConn3 -- Spring/LConn2
  R2/RConn1 -- SuspA2/RConn3
  L2/RConn1 -- SuspA2/LConn2
  Tire R2/RConn1 -- SuspA2/RConn2
  SuspA2/LConn1 -- Tire L2/RConn1
  SuspA1/RConn5 -- Damper/RConn1
  SuspA1/LConn4 -- Damper/LConn1
  SuspA1/RConn4 -- Spring/RConn1
  SuspA1/LConn3 -- Spring/LConn1
  Body/RConn1 -- SuspA1/RConn1 -- A1/RConn1
  Tire L1/RConn1 -- SuspA1/LConn1
  SuspA1/RConn2 -- Tire R1/RConn1
  SuspA1/RConn3 -- R1/RConn1
  SuspA1/LConn2 -- L1/RConn1
  A2/RConn1 -- Body/RConn2 -- SuspA2/RConn1
  W/RConn1 -- Aero/RConn1 -- Body/LConn3
  HitchF/RConn1 -- Body/LConn1

== system sm_car/Vehicle/Vehicle/Powertrain ==
  CtrlD : Inport
  CtrlP : Inport  Port=2
  VehB : Inport  Port=3
  Driveline : Subsystem  Tag=PublishSubsystem  Variant=on  VariantControlMode=label  VariantControl=Shaft  LabelModeActiveChoice=L1_R1_L2_R2  mask(Variants for Driveline){Driveline=Powertrain.Driveline, VariantLabel=Powertrain.Driveline.class.Value}
      mask prompts: Driveline "Driveline Parameters"; VariantLabel "Variant Label"
      mask help: Select option and provide parameters for driveline. Option is chosen by string provided in Variant Label. The parameters for the selected option are contained in Driveline data structure.
      mask init:
      | curblk = gcb;
      | 
      | % Set variant for this block 
      | set_param(curblk,'LabelModeActiveChoice',VariantLabel);
      settings: AttributesFormatString=%<ActiveVariant>
      mask Help: web('sm_car_doc_driveline.html');
  Power : Subsystem  Variant=on  VariantControlMode=label  VariantControl=Variant1  LabelModeActiveChoice=Electric_L1_R1_L2_R2  mask(Variants for Power){Power=Powertrain.Power, VariantLabel=Powertrain.Power.class.Value}
      mask prompts: Power "Power Parameters"; VariantLabel "Variant Label"
      mask help: Select option and provide parameters for power system (energy storage and actuator). Option is chosen by string provided in Variant Label. The parameters for the selected option are contained in Power data structure.
      mask init:
      | curblk = gcb;
      | 
      | % Set variant for this block 
      | set_param(curblk,'LabelModeActiveChoice',VariantLabel);
      settings: AttributesFormatString=%<ActiveVariant>
  FA : PMIOPort  Side=Left
  Ref : PMIOPort  Port=2  Side=Right
  RA : PMIOPort  Port=3  Side=Right
  R1 : PMIOPort  Port=4  Side=Right
  L1 : PMIOPort  Port=5  Side=Left
  L2 : PMIOPort  Port=6  Side=Left
  R2 : PMIOPort  Port=7  Side=Right
  OutD : Outport  VectorParamsAs1DForOutWhenUnconnected=off
  OutP : Outport  Port=2  VectorParamsAs1DForOutWhenUnconnected=off
  wires:
  Driveline/1(OutD) -> OutD/1
  CtrlD/1 -> Driveline/1(CtrlBus)
  Power/1(OutP) -> OutP/1
  CtrlP/1 -> Power/1(CtrlBus)
  VehB/1 -> Power/2(VehBus)
  connections:
  Driveline/LConn1 -- FA/RConn1
  Ref/RConn1 -- Power/RConn1
  Driveline/RConn1 -- RA/RConn1
  Driveline/LConn4 -- Power/LConn1
  Driveline/LConn2 -- L1/RConn1
  Driveline/RConn2 -- R1/RConn1
  Driveline/RConn3 -- R2/RConn1
  Driveline/LConn3 -- L2/RConn1

== system sm_car/Vehicle/Vehicle/Wheel Spin ==
  Free : Subsystem  VariantControl=Free
  L1 : PMIOPort  Side=Left
  L2 : PMIOPort  Port=2  Side=Left
  R1 : PMIOPort  Port=3  Side=Right
  R2 : PMIOPort  Port=4  Side=Right

== system sm_car/Vehicle/Vehicle Constraint/No Constraint ==
  F : PMIOPort  Side=Right
  B : PMIOPort  Port=2  Side=Left

== system sm_car/Visualization/Unreal/Animation Off ==
  xyz : Inport
  rpy : Inport  Port=2
  ws : Inport  Port=3
  aCamber : Inport  Port=4
  aSteerWheel : Inport  Port=5
  Terminator{,1..4} (5 alike) : Terminator
  wires:
  rpy/1 -> Terminator1/1
  aSteerWheel/1 -> Terminator4/1
  aCamber/1 -> Terminator3/1
  xyz/1 -> Terminator/1
  ws/1 -> Terminator2/1

== system sm_car/World/Mechanism Configuration/Constant Gravity ==
  MechanismConfiguration : sm_lib/Utilities/Mechanism Configuration  UniformGravity=Constant  GravityVector=GravityVector  GravityVectorUnits=m/s^2  LinearizationDelta=0.001  JointModeTransitionNonlinearIterations=2
  C : PMIOPort  Side=Right
  connections:
  MechanismConfiguration/RConn1 -- C/RConn1
